simulink model "sschdlexThreePhaseRectifierModel"  (R2026a)
settings: Solver=FixedStepDiscrete  StopTime=0.025  RelTol=1e-6  AbsTol=1e-6
libraries: fl_lib x13, nesl_utility x11, ee_lib x6
settings Model: DataTypeOverride=Off  Creator=The MathWorks, Inc.  LastModifiedBy=The MathWorks, Inc.
settings OptimizationCC: ConditionallyExecuteInputs=off
settings DebuggingCC: AlgebraicLoopMsg=error  SingleTaskRateTransMsg=error  PregeneratedLibrarySubsystemCodeDiagnostic=none
settings HardwareCC: ProdHWDeviceType=ASIC/FPGA->ASIC/FPGA  TargetBitPerLong=64.0  TargetBitPerPointer=64.0  TargetBitPerSizeT=64.0  TargetBitPerPtrDiffT=64.0  TargetLongLongMode=on  TargetIntDivRoundTo=Zero  TargetEndianess=LittleEndian  TargetWordSize=64.0  TargetHWDeviceType=Custom Processor->MATLAB Host Computer  ProdEqTarget=off
settings SimscapeCC: SimscapeNormalizeSystem=off  SimscapeNominalValues="[{\"value\":\"10\",\"unit\":\"V\"},{\"value\":\"1\",\"unit\":\"A\"},{\"value\":\"10\",\"unit\":\"N*m\"},{\"value\":\"10\",\"unit\":\"bar\"},{\"value\":\"100\",\"unit\":\"kJ/kg\"},{\"value\":\"1\",\"unit\":\"kW\"},{\"value\":\"300\",\"unit\":\"K\"},{\"value\":\"100\",\"unit\":\"cm^3/s\"},{\"value\":\"1\",\"unit\":\"kN\"},{\"value\":\"1\",\"unit\":\"g/cm^3\"},{\"value\":\"1\",\"unit\":\"l\"},{\"value\":\"1\",\"unit\":\"cm^2\"},{\"value\":\"60\",\"unit\":\"Hz\"}]"

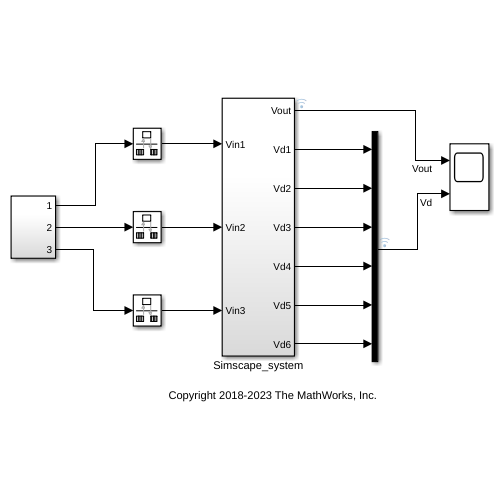
[thumbnail: Simulink's stored preview of the top-level diagram]
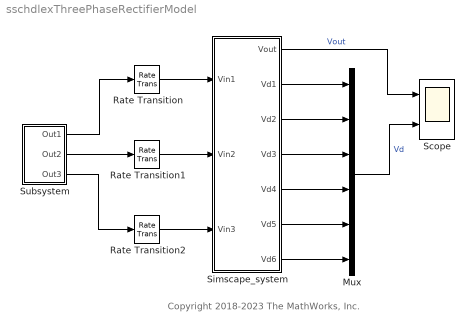
== system sschdlexThreePhaseRectifierModel ==
  note: Copyright 2018-2023 The MathWorks, Inc.
  Mux : Mux  Inputs=6
  Rate Transition : RateTransition
  Rate Transition1 : RateTransition
  Rate Transition2 : RateTransition
  Scope : Scope  NumInputPorts=2
      settings: ActiveDisplayYMinimum=-125  ActiveDisplayYMaximum=125
  Simscape_system : Subsystem
  Subsystem : Subsystem
  wires:
  Simscape_system/2(Vd1) -> Mux/1
  Simscape_system/3(Vd2) -> Mux/2
  Simscape_system/4(Vd3) -> Mux/3
  Simscape_system/5(Vd4) -> Mux/4
  Simscape_system/6(Vd5) -> Mux/5
  Simscape_system/7(Vd6) -> Mux/6
  Subsystem/1(Out1) -> Rate Transition/1
  Subsystem/2(Out2) -> Rate Transition1/1
  Subsystem/3(Out3) -> Rate Transition2/1
  Rate Transition/1 -> Simscape_system/1(Vin1)
  Rate Transition1/1 -> Simscape_system/2(Vin2)
  Rate Transition2/1 -> Simscape_system/3(Vin3)
  Simscape_system/1(Vout) -> Scope/1  "Vout"
  Mux/1 -> Scope/2  "Vd"

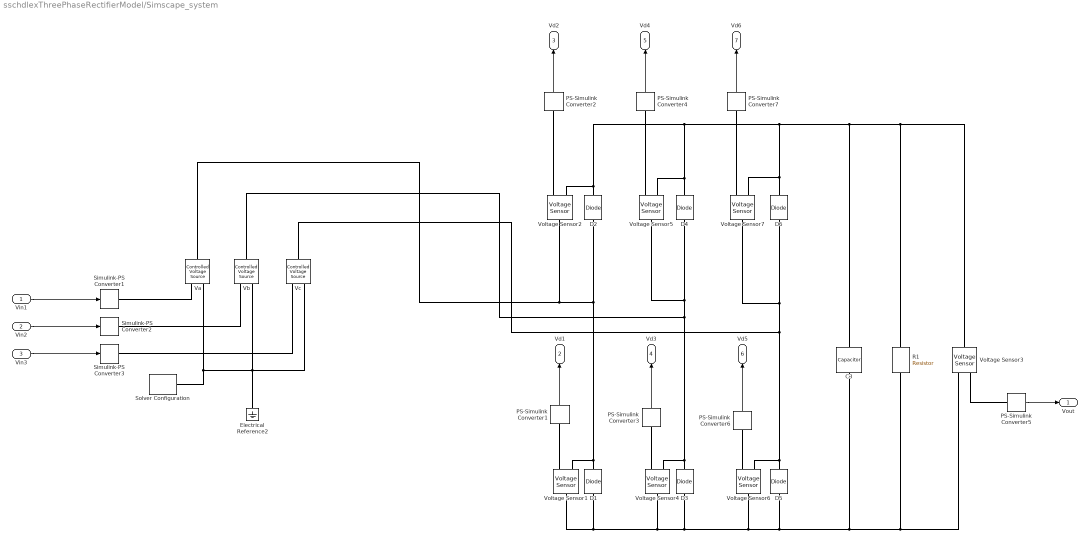
== system sschdlexThreePhaseRectifierModel/Simscape_system ==
  Vin1 : Inport
  Vin2 : Inport  Port=2
  Vin3 : Inport  Port=3
  C3 : fl_lib/Electrical/Electrical Elements/Capacitor  c=10e-3 F  r=1e-6 Ohm  g=0 1/Ohm  i_specify=off  i_priority=None  i=0 A  i_nominal_specify=off  i_nominal_value=1  i_nominal_unit=A  v_specify=off  v_priority=None  v=0 V  v_nominal_specify=off  v_nominal_value=1  v_nominal_unit=V  vc_specify=on  vc_priority=High  vc=150 V  vc_nominal_specify=off  vc_nominal_value=1  vc_nominal_unit=V
  D{1..6} (6 alike) : ee_lib/Semiconductors & Converters/Diode  ModelType=ee.enum.diode.modelType.pwl  TableType=ee.enum.diode.tableType.IfMat  IfMat=[.07, .12, .19, 1.75, 4.24, 7.32, 11.2; .16, .3, .72, 2.14, 5.02, 8.35, 13.12] A  VfMat=[.9, 1.15, 1.25, 1.5, 1.75, 2.17, 2.6, 2.85; .58, .68, .75, 1.1, 1.38, 1.77, 2.27, 2.7] V  TjVec=[25, 125] degC  VfVec=[.5, .7, .9, 1.3, 1.7, 2.1, 2.5] V  IfVec=[.1, .2, .5, 1, 2, 4, 7, 10] A  IrMat=[1e-06, 2e-06, 5e-06, 1e-05, 2.5e-05, 5e-05, .0001; 2e-06, 5e-06, 1e-05, 4e-05, 8e-05, .0002, .0005] A  VrMat=[10, 100, 200, 250, 300, 325, 350; 10, 70, 160, 220, 270, 300, 320] V  VrVec=[10, 20, 40, 50, 70, 80, 100] V  IrVec=[1e-06, 2e-06, 5e-06, 1e-05, 2e-05, 5e-05, .0001] A  Vf=0.8 V  Ron=0.001 Ohm  Goff=1e-5 S  prmExp=ee.enum.diode.expParam.useTwo  I12=[.0137, .545] A  V12=[.6, .7] V  RS=0 Ohm  Tmeas=25 degC  IS=1e-12 A  ec=1  I1=0.0137 A  V1=0.6 V  N_series=1  N_parallel=1  ZenerEnable=false  Rz=0.3 Ohm  BV=inf V  C_param=ee.enum.diode.capParam.fixed  CJ=0 pF  CJ0=5 pF  Vvec=[.1, 10, 100] V  Cvec=[3.5, 1, .4] pF  VJ=1 V  Mgrad=0.5  FC=0.5  Q_param=ee.enum.diode.recoveryParam.off  iRM=-7.15 A  iF=4 A  didt=-750 A/us  trr_factor=3  trr=115 ns  Qrr=150 nA*s  Vr=-600 V  Ls=150 nH  Erec=0.03 J  TT=50 ns  tau=100 ns  T_param=ee.enum.diode.temperatureParam.off  Tdevice=25 degC  I1_T2=0.245 A  V1_T2=0.5 V  IS_T2=1.25e-7 A  Tmeas2=125 degC  XTI_param=ee.enum.diode.xtiParam.pn  XTI=3  EG_param=ee.enum.diode.egapParam.material_si  EG=1.11 eV  dBVdT=0 V/K  enable_fault_input=simscape.enum.onoff.off  i_specify=off  i_priority=None  i=0 A  i_nominal_specify=off  i_nominal_value=1  i_nominal_unit=A  v_specify=off  v_priority=None  v=0 V  v_nominal_specify=off  v_nominal_value=1  v_nominal_unit=V  v_capacitor_specify=off  v_capacitor_priority=None  v_capacitor=0 V  v_capacitor_nominal_specify=off  v_capacitor_nominal_value=1  v_capacitor_nominal_unit=V  Qj_specify=off  Qj_priority=High  Qj=0 C  Qj_nominal_specify=off  Qj_nominal_value=1  Qj_nominal_unit=C  i_diode_specify=off  i_diode_priority=None  i_diode=0 A  i_diode_nominal_specify=off  i_diode_nominal_value=1  i_diode_nominal_unit=A  v_diode_specify=off  v_diode_priority=None  v_diode=0 V  v_diode_nominal_specify=off  v_diode_nominal_value=1  v_diode_nominal_unit=V  i_capacitor_specify=off  i_capacitor_priority=None  i_capacitor=0 A  i_capacitor_nominal_specify=off  i_capacitor_nominal_value=1  i_capacitor_nominal_unit=A  fidelity_level=ee.enum.diode.fidelity.includeChargeDyn  rec_loss_model=ee.enum.diode.reverseRecoveryModel.fixed  ErecVal=0 J  scaleWithIandV=true  ErecMat=zeros(2, 3) J  ErecMat3D=zeros(2, 3, 2) J  TjrecVec=[298.15, 398.15] K  IfrecVec=[.1, 1, 10] A  IrecVal=10 A  VrecVal=10 V  VrecVec=[0, 100] V  tFilter=1 / 1000 / 100 s  thermal_network_parameterization=ee.enum.thermalNetworkTopology.junctionCase  Rth=[0, 10] K/W  Rth_Cauer=[1, 3, 10] K/W  Rth_Foster=[4, 6] K/W  thermal_mass_parameterization=ee.enum.thermalNetwork.timeconstant  thermal_mass=[0, 1] J/K  thermal_mass_Cauer=[.1, .3, 1] J/K  thermal_mass_Foster=[1.5, 3] J/K  thermal_time_constant=[0, 10] s  thermal_time_constant_Cauer=[1, 3, 10] s  thermal_time_constant_Foster=[6, 18] s  thermal_mass_initial_temperatures=[25, 25] degC  thermal_mass_initial_temperatures_Cauer=[25, 25, 25] degC  junction_thermal_mass=0.01 J/K  Tvec_initial_Foster=[25, 25, 25, 25] degC  no_thermal_network=0  junction_temperature_specify=off  junction_temperature_priority=None  junction_temperature=25 degC  junction_temperature_nominal_specify=off  junction_temperature_nominal_value=1  junction_temperature_nominal_unit=degC
  Electrical Reference2 : fl_lib/Electrical/Electrical Elements/Electrical Reference
  PS-Simulink Converter{1..7} (7 alike) : nesl_utility/PS-Simulink Converter  PhysicalDomain=network_engine_domain  SubClassName=ps_output  LeftPortType=input  RightPortType=output  PseudoPeriodic=off  Frequencies=[]  VectorFormat=1-D array  Unit=1  AffineConversion=off
  R1 : fl_lib/Electrical/Electrical Elements/Resistor  R=1 Ohm  i_specify=off  i_priority=None  i=0 A  i_nominal_specify=off  i_nominal_value=1  i_nominal_unit=A  v_specify=off  v_priority=None  v=0 V  v_nominal_specify=off  v_nominal_value=1  v_nominal_unit=V
  Simulink-PS Converter1 : nesl_utility/Simulink-PS Converter  PhysicalDomain=network_engine_domain  SubClassName=ps_input  LeftPortType=input  RightPortType=output  PseudoPeriodic=off  Frequencies=[]  NoiseDistribution=none  NoiseParameters=[]  Unit=1  AffineConversion=off  FilteringAndDerivatives=zero  SimscapeFilterOrder=1  InputFilterTimeConstant=0.001  UdotUserProvided=1
  Simulink-PS Converter2 : nesl_utility/Simulink-PS Converter  PhysicalDomain=network_engine_domain  SubClassName=ps_input  LeftPortType=input  RightPortType=output  PseudoPeriodic=off  Frequencies=[]  NoiseDistribution=none  NoiseParameters=[]  Unit=1  AffineConversion=off  FilteringAndDerivatives=zero  SimscapeFilterOrder=1  InputFilterTimeConstant=0.001  UdotUserProvided=1
  Simulink-PS Converter3 : nesl_utility/Simulink-PS Converter  PhysicalDomain=network_engine_domain  SubClassName=ps_input  LeftPortType=input  RightPortType=output  PseudoPeriodic=off  Frequencies=[]  NoiseDistribution=none  NoiseParameters=[]  Unit=1  AffineConversion=off  FilteringAndDerivatives=zero  SimscapeFilterOrder=1  InputFilterTimeConstant=0.001  UdotUserProvided=1
  Solver Configuration : nesl_utility/Solver Configuration  PhysicalDomain=network_engine_domain  SubClassName=solver  LeftPortType=input  RightPortType=generic  Tones=[]  Harmonics=[]  SimulateNoise=off  Profile=off  UseLocalSampling=off  EnableSwitchedLinearOptims=on  FrequencyDomain=off  UseCCode=off  RelTol=0.001  AbsTol=1e-06  MinStep=1e-09  ToWorkspace=off  RevertToSquareIcSolve=off  NumHomotopyIterations=100  PhasorMode=off  PhasorModeNumHarmonics=1  ConsistencySolver=NEWTON_FTOL  CanonicalOrdering=UNORDERED  OptimizeIntermediates=UNOPTIMIZED  IndexReductionMethod=DerivativeReplacement  DoDC=off  ResidualTolerance=1e-09  ConsistencyTolSource=GLOBAL  ConsistencyAbsTol=0.001  ConsistencyRelTol=0.001  ConsistencyTolFactor=0.001  UseLocalSolver=on  LocalSolverChoice=NE_BACKWARD_EULER_ADVANCER  ResolveIndetEquations=on  FunctionEvalNumThread=1  LocalSolverSampleTime=1e-05  DoFixedCost=off  MaxNonlinIter=3  MaxModeIter=2  ComputeImpulses=off  ImpulseIterations=2  LinearAlgebra=Sparse  LinearAlgebraNumThread=0  EquationFormulation=NE_TIME_EF  DelaysMemoryBudget=1024  AutomaticFiltering=on  FilteringTimeConstant=0.001  PartitionStorageMethod=AS_NEEDED  PartitionMemoryBudget=1024  PartitionMethod=FAST  MultibodyUseLocalSolver=off  MultibodyLocalSolverChoice=ODE1  MultibodyLocalSolverSampleTime=0.001
  Va : fl_lib/Electrical/Electrical Sources/Controlled Voltage Source
  Vb : fl_lib/Electrical/Electrical Sources/Controlled Voltage Source
  Vc : fl_lib/Electrical/Electrical Sources/Controlled Voltage Source
  Voltage Sensor{1..7} (7 alike) : fl_lib/Electrical/Electrical Sensors/Voltage Sensor
  Vout : Outport  VectorParamsAs1DForOutWhenUnconnected=off
  Vd1 : Outport  Port=2  VectorParamsAs1DForOutWhenUnconnected=off
  Vd2 : Outport  Port=3  VectorParamsAs1DForOutWhenUnconnected=off
  Vd3 : Outport  Port=4  VectorParamsAs1DForOutWhenUnconnected=off
  Vd4 : Outport  Port=5  VectorParamsAs1DForOutWhenUnconnected=off
  Vd5 : Outport  Port=6  VectorParamsAs1DForOutWhenUnconnected=off
  Vd6 : Outport  Port=7  VectorParamsAs1DForOutWhenUnconnected=off
  wires:
  PS-Simulink Converter5/1 -> Vout/1
  PS-Simulink Converter2/1 -> Vd2/1
  PS-Simulink Converter1/1 -> Vd1/1
  PS-Simulink Converter3/1 -> Vd3/1
  PS-Simulink Converter4/1 -> Vd4/1
  PS-Simulink Converter6/1 -> Vd5/1
  Vin2/1 -> Simulink-PS Converter2/1
  Vin3/1 -> Simulink-PS Converter3/1
  Vin1/1 -> Simulink-PS Converter1/1
  PS-Simulink Converter7/1 -> Vd6/1
  connections:
  PS-Simulink Converter2/LConn1 -- Voltage Sensor2/RConn1
  Vc/LConn1 -- D6/LConn1 -- Voltage Sensor7/LConn1 -- D5/RConn1 -- Voltage Sensor6/RConn2
  Voltage Sensor6/LConn1 -- D3/LConn1 -- D1/LConn1 -- Voltage Sensor1/LConn1 -- Voltage Sensor4/LConn1 -- D5/LConn1 -- R1/RConn1 -- Voltage Sensor3/RConn2 -- C3/RConn1
  Va/LConn1 -- Voltage Sensor2/LConn1 -- D2/LConn1 -- D1/RConn1 -- Voltage Sensor1/RConn2
  C3/LConn1 -- R1/LConn1 -- Voltage Sensor3/LConn1 -- D6/RConn1 -- Voltage Sensor7/RConn2 -- D2/RConn1 -- Voltage Sensor2/RConn2 -- D4/RConn1 -- Voltage Sensor5/RConn2
  PS-Simulink Converter5/LConn1 -- Voltage Sensor3/RConn1
  Va/RConn2 -- Electrical Reference2/LConn1 -- Vb/RConn2 -- Vc/RConn2 -- Solver Configuration/RConn1
  Voltage Sensor5/LConn1 -- D4/LConn1 -- Vb/LConn1 -- D3/RConn1 -- Voltage Sensor4/RConn2
  PS-Simulink Converter1/LConn1 -- Voltage Sensor1/RConn1
  PS-Simulink Converter3/LConn1 -- Voltage Sensor4/RConn1
  PS-Simulink Converter4/LConn1 -- Voltage Sensor5/RConn1
  PS-Simulink Converter6/LConn1 -- Voltage Sensor6/RConn1
  PS-Simulink Converter7/LConn1 -- Voltage Sensor7/RConn1
  Simulink-PS Converter3/RConn1 -- Vc/RConn1
  Simulink-PS Converter2/RConn1 -- Vb/RConn1
  Simulink-PS Converter1/RConn1 -- Va/RConn1

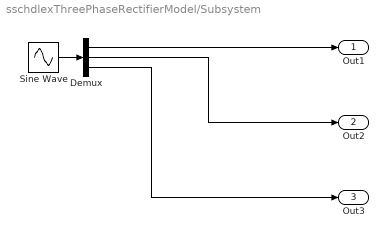
== system sschdlexThreePhaseRectifierModel/Subsystem ==
  Demux : Demux  Outputs=3
  Sine Wave : Sin  Amplitude=100  Frequency=60*2*pi  Phase=[0 -2*pi/3 2*pi/3]  SampleTime=0
  Out1 : Outport  VectorParamsAs1DForOutWhenUnconnected=off
  Out2 : Outport  Port=2  VectorParamsAs1DForOutWhenUnconnected=off
  Out3 : Outport  Port=3  VectorParamsAs1DForOutWhenUnconnected=off
  wires:
  Sine Wave/1 -> Demux/1
  Demux/1 -> Out1/1
  Demux/2 -> Out2/1
  Demux/3 -> Out3/1
